simulink model "lab1"  (R2012b)
settings: Solver=ode45  StartTime=0.0  StopTime=10.0  RelTol=1e-3
undefined symbols (not defined in the file): des, gcbh
settings Model: Creator=Student  LastModifiedBy=Student

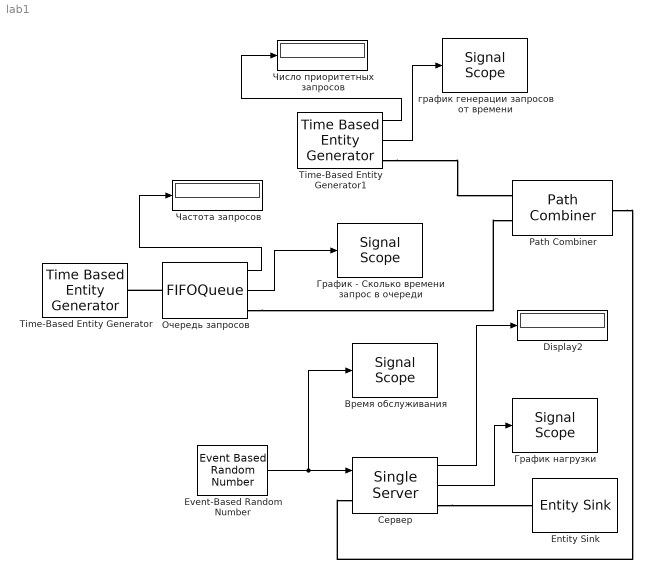
== system lab1 ==
  Display2 : Display
  Entity Sink : EntitySink
  Event-Based Random Number : EventBasedRandomNumber  Distribution=Uniform  minUnif=1  maxUnif=2  Seed=1234
  Path Combiner : PathCombiner  NumberInputPorts=2
  Time-Based Entity Generator : TimeBasedEntityGenerator  Period=2
  Time-Based Entity Generator1 : TimeBasedEntityGenerator  Period=10  StatNumberDeparted=on  StatAverageIntergenerationTime=on
      settings: OutputPortMap=o0,o2
  Время обслуживания : SignalScope  LoadFcn=des.scope.CallbackSupport('seLoadFcn',gcbh)  StartFcn=des.scope.CallbackSupport('seStartFcn',gcbh)  StopFcn=des.scope.CallbackSupport('seStopFcn',gcbh)
      settings: CopyFcn=des.scope.CallbackSupport('seCopyFcn',gcbh)  DeleteFcn=des.scope.CallbackSupport('seDeleteFcn',gcbh)  PreSaveFcn=des.scope.CallbackSupport('sePreSaveFcn',gcbh)  NameChangeFcn=des.scope.CallbackSupport('seNameChangeFcn',gcbh)  OpenFcn=des.scope.CallbackSupport('seOpenFcn',gcbh)
  График - Сколько времени запрос в очереди : SignalScope  LoadFcn=des.scope.CallbackSupport('seLoadFcn',gcbh)  StartFcn=des.scope.CallbackSupport('seStartFcn',gcbh)  StopFcn=des.scope.CallbackSupport('seStopFcn',gcbh)
      settings: CopyFcn=des.scope.CallbackSupport('seCopyFcn',gcbh)  DeleteFcn=des.scope.CallbackSupport('seDeleteFcn',gcbh)  PreSaveFcn=des.scope.CallbackSupport('sePreSaveFcn',gcbh)  NameChangeFcn=des.scope.CallbackSupport('seNameChangeFcn',gcbh)  OpenFcn=des.scope.CallbackSupport('seOpenFcn',gcbh)
  График нагрузки : SignalScope  LoadFcn=des.scope.CallbackSupport('seLoadFcn',gcbh)  StartFcn=des.scope.CallbackSupport('seStartFcn',gcbh)  StopFcn=des.scope.CallbackSupport('seStopFcn',gcbh)
      settings: CopyFcn=des.scope.CallbackSupport('seCopyFcn',gcbh)  DeleteFcn=des.scope.CallbackSupport('seDeleteFcn',gcbh)  PreSaveFcn=des.scope.CallbackSupport('sePreSaveFcn',gcbh)  NameChangeFcn=des.scope.CallbackSupport('seNameChangeFcn',gcbh)  OpenFcn=des.scope.CallbackSupport('seOpenFcn',gcbh)
  Очередь запросов : FIFOQueue  StatNumberDeparted=on  StatAverageWait=on
      settings: OutputPortMap=o0,o2
  Сервер : SingleServer  ServiceTimeFrom=Signal port t  StatNumberDeparted=on  StatUtilization=on
      settings: OutputPortMap=o0,o5
  "Частота запросов " : Display
  "Число приоритетных запросов " : Display
  график генерации запросов от времени : SignalScope  LoadFcn=des.scope.CallbackSupport('seLoadFcn',gcbh)  StartFcn=des.scope.CallbackSupport('seStartFcn',gcbh)  StopFcn=des.scope.CallbackSupport('seStopFcn',gcbh)
      settings: CopyFcn=des.scope.CallbackSupport('seCopyFcn',gcbh)  DeleteFcn=des.scope.CallbackSupport('seDeleteFcn',gcbh)  PreSaveFcn=des.scope.CallbackSupport('sePreSaveFcn',gcbh)  NameChangeFcn=des.scope.CallbackSupport('seNameChangeFcn',gcbh)  OpenFcn=des.scope.CallbackSupport('seOpenFcn',gcbh)
  wires:
  Очередь запросов/1 -> "Частота запросов "/1
  Очередь запросов/2 -> График - Сколько времени запрос в очереди/1
  Time-Based Entity Generator1/2 -> график генерации запросов от времени/1
  Time-Based Entity Generator1/1 -> "Число приоритетных запросов "/1
  Event-Based Random Number/1 -> Сервер/1, Время обслуживания/1
  Сервер/1 -> Display2/1
  Сервер/2 -> График нагрузки/1
  connections:
  Очередь запросов/LConn1 -- Time-Based Entity Generator/RConn1
  Очередь запросов/RConn1 -- Path Combiner/LConn2
  Time-Based Entity Generator1/RConn1 -- Path Combiner/LConn1
  Сервер/RConn1 -- Entity Sink/LConn1
  Path Combiner/RConn1 -- Сервер/LConn1
